simulink model "scheme_L2"  (R2026b)
settings: Solver=VariableStepAuto
settings Model: Creator=yzhar  LastModifiedBy=Dmitrii
settings RTWCC: GPUComputeCapability=5.0

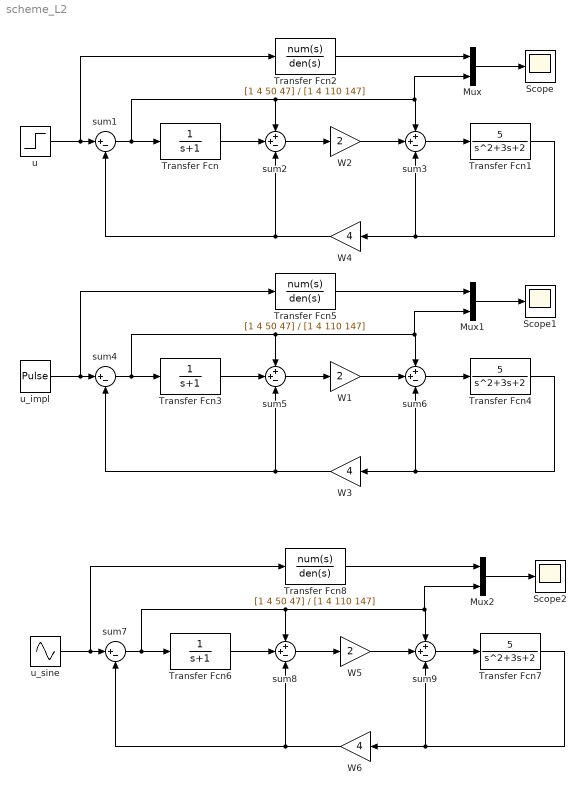
== system scheme_L2 ==
  Mux : Mux  Inputs=2
  Mux1 : Mux  Inputs=2
  Mux2 : Mux  Inputs=2
  Scope : Scope
      settings: ActiveDisplayYMinimum=-0.12499999999999997  ActiveDisplayYMaximum=1.125
  Scope1 : Scope
      settings: ActiveDisplayYMinimum=-3.2668344830119445  ActiveDisplayYMaximum=4.6991453957452354
  Scope2 : Scope
      settings: ActiveDisplayYMinimum=-0.45316380038683146  ActiveDisplayYMaximum=0.45386123588739152  DataLoggingVariableName=ScopeData2
  Transfer Fcn : TransferFcn  Denominator=[1 1]
  Transfer Fcn1 : TransferFcn  Numerator=[5]  Denominator=[1 3 2]
  Transfer Fcn2 : TransferFcn  Numerator=[1 4 50 47]  Denominator=[1 4 110 147]
  Transfer Fcn3 : TransferFcn  Denominator=[1 1]
  Transfer Fcn4 : TransferFcn  Numerator=[5]  Denominator=[1 3 2]
  Transfer Fcn5 : TransferFcn  Numerator=[1 4 50 47]  Denominator=[1 4 110 147]
  Transfer Fcn6 : TransferFcn  Denominator=[1 1]
  Transfer Fcn7 : TransferFcn  Numerator=[5]  Denominator=[1 3 2]
  Transfer Fcn8 : TransferFcn  Numerator=[1 4 50 47]  Denominator=[1 4 110 147]
  W1 : Gain  Gain=2
  W2 : Gain  Gain=2
  W3 : Gain  Gain=4
  W4 : Gain  Gain=4
  W5 : Gain  Gain=2
  W6 : Gain  Gain=4
  sum1 : Sum  Inputs=|+-
  sum{2..3,5..6,8..9} (6 alike) : Sum  Inputs=++-
  sum4 : Sum  Inputs=|+-
  sum7 : Sum  Inputs=|+-
  u : Step  SampleTime=0
  u_impl : DiscretePulseGenerator  PulseType=Time based  Period=10  PulseWidth=5
  u_sine : Sin  SampleTime=0
  wires:
  u/1 -> Transfer Fcn2/1, sum1/1
  sum1/1 -> Transfer Fcn/1, sum3/1, Mux/2, sum2/1
  Transfer Fcn/1 -> sum2/2
  sum2/1 -> W2/1
  W2/1 -> sum3/2
  sum3/1 -> Transfer Fcn1/1
  Transfer Fcn1/1 -> sum3/3, W4/1
  W4/1 -> sum2/3, sum1/2
  Transfer Fcn2/1 -> Mux/1
  Mux/1 -> Scope/1
  u_impl/1 -> Transfer Fcn5/1, sum4/1
  W1/1 -> sum6/2
  Transfer Fcn3/1 -> sum5/2
  W3/1 -> sum5/3, sum4/2
  sum6/1 -> Transfer Fcn4/1
  Transfer Fcn4/1 -> sum6/3, W3/1
  Transfer Fcn5/1 -> Mux1/1
  sum4/1 -> Transfer Fcn3/1, sum6/1, Mux1/2, sum5/1
  sum5/1 -> W1/1
  Mux1/1 -> Scope1/1
  u_sine/1 -> Transfer Fcn8/1, sum7/1
  W5/1 -> sum9/2
  Transfer Fcn6/1 -> sum8/2
  W6/1 -> sum8/3, sum7/2
  sum9/1 -> Transfer Fcn7/1
  Transfer Fcn7/1 -> sum9/3, W6/1
  Transfer Fcn8/1 -> Mux2/1
  sum7/1 -> Transfer Fcn6/1, sum9/1, Mux2/2, sum8/1
  sum8/1 -> W5/1
  Mux2/1 -> Scope2/1
